simulink model "ASM_Traffic_new"  (R2024a)
settings: Solver=ode1  StartTime=SIM.tstart.v  StopTime=SIM.tend.v  FixedStep=SIM.StepSize.v  RelTol=1e-3
PostLoadFcn:
  | if any(exist('dsrtsu_mdlpostloadfcn', 'file') ~= 0), dsrtsu_mdlpostloadfcn('Execute', bdroot); end
  | try, asm_mdl_postloadfcn(bdroot, 'UpdateModel', 3600); catch, disp(lasterr); end,
InitFcn:
  | , if any(exist('rtifpga_mdlclblib', 'file') ~= 0), rtifpga_mdlclblib('Init', bdroot); end,
  | , if any(exist('dsmpb_private', 'file') ~= 0), dsmpb_private('dsmpb_mdlclblib', 'Init', bdroot); end,
undefined symbols (not defined in the file): _to_, a0b2, ASM_BrakeHydraulics_DemoSystems, ASM_VehicleDynamics_DemoSystems, b98103fe8ad365046cd0, BrakeCircuit, CPT, Crankshaft, DiscIntNeverNeededParam, dsmsi, FinalDriveAssembly, MDL, ModeSignals, Pos_BrakePedal_Maneuver, rad, RefSignals, s_to_rpm, SIM, SoftECU, Suspension, Tire, Transmission
libraries: ASM_Traffic_lib x135, simulink x100, ASM_Utils_lib x77, ASM_VehicleDynamics_lib x70, ASM_Environment_lib x22, dsmpblib x20, dsmsilib x15, MDLD_Utils_lib x10, ASM_BrakeHydraulics_lib x3
(part 5 of 63)

== system ASM_Traffic_new/VehicleDynamics/Interface_In ==
  note: Vehicle Dynamics
  In : Inport
  Bus Creator2 : BusCreator  Inputs=3
  Bus Selector : BusSelector  OutputSignals=Environment.Plant.Sw_ModelPortBlocks[0Disabled|1Enabled],Environment.Plant.Sw_ModelDeskPlottingInterface[0Disabled|1Enabled],Engine.Plant.Trq_MeanEff_Engine[Nm],Driver.Plant.Pos_BrakePedal[%],Driver.Plant.Pos_AccPedal[%],Environment.Plant.Reset_States[0|1],Environment.Plant.ECU_Commands[],DomainControl.TorqueManager.Control.Vehicle_Topology[-2|-1|0|2],Drivetrain.Plant.Trq_Shaft[FL;FR;RL;RR][Nm],Environment.Plant.v_Wind_Coor_Sys_E[x;y;z][m|s],Environment.Plant.p_Ambient[Pa],Environment.Plant.T_Ambient[degC],Driver.Plant.Angle_SteeringWheel[deg],Environment.Plant.Trq_Driver_External[Nm],Environment.Plant.Pos_z_CP[:][m],Environment.Plant.Fric_Coeff_CP[:][],Environment.Plant.UnitVec_z_CP[:][x;y;z],Environment.Plant.Sw_Tire_Parameter_Set_CP[:][1|2|3|4],Environment.Plant.Sw_ParkingBrake[0Off|1On],Environment.Plant.Sw_SteeringMode[1Angle|2Trq],Environment.Plant.Keep_VehiclePosition[0|1],Environment.Plant.Pos_Vehicle_Init_CoorSys_E[x;y;z][m],Environment.Plant.Angle_Vehicle_Init_CoorSys_E[x;y;z][rad],Environment.Plant.q_dt_Vehicle_Init[6x1],Environment.Plant.Sw_Steering_Mode[1Manual|2ManSched],Environment.Plant.Const_Steering_Mode_Manual[1Angle|2Trq],DomainControl.StartSystem.Control.Sw_Ignition[0|1],DomainControl.DriverAssistance.Control.Enable_Trq_Decrease_ACC[0|1],DomainControl.DriverAssistance.Control.Trq_DecreaseRequest_ACC[Nm],DomainControl.TorqueManager.Control.Trq_Request_Brake[Nm]
  Bus Selector1 : BusSelector  OutputSignals=Environment.Plant.Sw_ModelPortBlocks[0Disabled|1Enabled]
  ExternalSignals : Subsystem
  M_Articulated_T[1x36] : Constant  Value=zeros(1,36)
  ModelSignals : Subsystem
  Q_Articulated_T[6x1] : Constant  Value=[0; 0; 0; 0; 0; 0]
  Trq[Nm] : Constant  Value=0
  Trq_Hitch_CoorSys_V[x;y;z][Nm] : Constant  Value=[0 0 0]
  Out : Outport  VectorParamsAs1DForOutWhenUnconnected=off
  wires:
  Bus Selector1/1 -> ExternalSignals/Enable  "<Sw_ModelPortBlocks[0Disabled|1Enabled]>"
  ExternalSignals/2(ExternalPlant) -> Bus Creator2/3
  ExternalSignals/1(ExternalECU) -> Bus Creator2/2
  Bus Creator2/1 -> Out/1
  ModelSignals/1(Out) -> Bus Creator2/1
  Trq[Nm]/1 -> ModelSignals/31(Trq_EM_Front[Nm])
  Q_Articulated_T[6x1]/1 -> ModelSignals/32(Q_Articulated_T[6x1])
  Trq_Hitch_CoorSys_V[x;y;z][Nm]/1 -> ModelSignals/33(Trq_Hitch_CoorSys_V[x;y;z][Nm])
  M_Articulated_T[1x36]/1 -> ModelSignals/34(M_Articulated_T[1x36])
  Bus Selector/1 -> ModelSignals/1(Sw_ModelPortBlocks[0Disabled|1Enabled])  "<Sw_ModelPortBlocks[0Disabled|1Enabled]>"
  Bus Selector/2 -> ModelSignals/2(Sw_ModelDeskPlottingInterface[0Disabled|1Enabled])  "<Sw_ModelDeskPlottingInterface[0Disabled|1Enabled]>"
  Bus Selector/3 -> ModelSignals/3(Trq_Eff_Engine[Nm])  "<Trq_MeanEff_Engine[Nm]>"
  Bus Selector/4 -> ModelSignals/4(Pos_BrakePedal[%])  "<Pos_BrakePedal[%]>"
  Bus Selector/5 -> ModelSignals/5(Pos_AccPedal[%])  "<Pos_AccPedal[%]>"
  Bus Selector/6 -> ModelSignals/6(Reset_VehicleStates[0|1])  "<Reset_States[0|1]>"
  Bus Selector/7 -> ModelSignals/7(ECU_Commands[])  "<ECU_Commands[]>"
  Bus Selector/8 -> ModelSignals/8(Vehicle_Topology[-2|-1|0|2])  "<Vehicle_Topology[-2|-1|0|2]>"
  Bus Selector/9 -> ModelSignals/9(Trq_Shaft[FL,FR,RL,RR][Nm])  "<Trq_Shaft[FL;FR;RL;RR][Nm]>"
  Bus Selector/10 -> ModelSignals/10(v_Wind_Coor_Sys_E[x;y;z][m|s])  "<v_Wind_Coor_Sys_E[x;y;z][m|s]>"
  Bus Selector/11 -> ModelSignals/11(p_Ambient[Pa])  "<p_Ambient[Pa]>"
  Bus Selector/12 -> ModelSignals/12(T_Ambient[degC])  "<T_Ambient[degC]>"
  Bus Selector/13 -> ModelSignals/13(Angle_SteeringWheel[deg])  "<Angle_SteeringWheel[deg]>"
  Bus Selector/14 -> ModelSignals/14(Trq_Driver_External[Nm])  "<Trq_Driver_External[Nm]>"
  Bus Selector/15 -> ModelSignals/15(Pos_z_CP[FL;FR;RL;RR][m])  "<Pos_z_CP[:][m]>"
  Bus Selector/16 -> ModelSignals/16(Fric_Coeff_CP[FL;FR;RL;RR][])  "<Fric_Coeff_CP[:][]>"
  Bus Selector/17 -> ModelSignals/17(UnitVec_z_CP[FL;FR;RL;RR][x;y;z])  "<UnitVec_z_CP[:][x;y;z]>"
  Bus Selector/18 -> ModelSignals/18(Sw_Tire_Parameter_Set_CP[FL;FR;RL;RR][1|2|3|4])  "<Sw_Tire_Parameter_Set_CP[:][1|2|3|4]>"
  Bus Selector/19 -> ModelSignals/19(Sw_ParkingBrake[0Off|1On])  "<Sw_ParkingBrake[0Off|1On]>"
  Bus Selector/20 -> ModelSignals/20(Sw_SteeringMode[1Angle|2Trq])  "<Sw_SteeringMode[1Angle|2Trq]>"
  Bus Selector/21 -> ModelSignals/21(Keep_VehiclePosition[0|1])  "<Keep_VehiclePosition[0|1]>"
  Bus Selector/22 -> ModelSignals/22(Pos_Vehicle_Init_CoorSys_E[x;y;z][m])  "<Pos_Vehicle_Init_CoorSys_E[x;y;z][m]>"
  Bus Selector/23 -> ModelSignals/23(Angle_Vehicle_Init_CoorSys_E[x;y;z][rad])  "<Angle_Vehicle_Init_CoorSys_E[x;y;z][rad]>"
  Bus Selector/24 -> ModelSignals/24(q_dt_Vehicle_Init[6x1])  "<q_dt_Vehicle_Init[6x1]>"
  Bus Selector/25 -> ModelSignals/25(Sw_Steering_Mode[1Manual|2ManSched])  "<Sw_Steering_Mode[1Manual|2ManSched]>"
  Bus Selector/26 -> ModelSignals/26(Const_Steering_Mode_Manual[1Angle|2Trq])  "<Const_Steering_Mode_Manual[1Angle|2Trq]>"
  Bus Selector/27 -> ModelSignals/27(Sw_Ignition[0Off|1On])  "<Sw_Ignition[0|1]>"
  Bus Selector/28 -> ModelSignals/28(Enable_Trq_Brake_Extern[0|1])  "<Enable_Trq_Decrease_ACC[0|1]>"
  Bus Selector/29 -> ModelSignals/29(Trq_Brake_Request_Extern[Nm])  "<Trq_DecreaseRequest_ACC[Nm]>"
  Bus Selector/30 -> ModelSignals/30(Trq_Request_Brake[Nm])  "<Trq_Request_Brake[Nm]>"
  In/1 -> Bus Selector/1, Bus Selector1/1

== system ASM_Traffic_new/VehicleDynamics/Interface_Out ==
  note: VehicleDynamics
  In : Inport
  Active_CP_VehDyn[] : Constant  Value=[1,2,3,4,5,6,9,10]
  Animation : Subsystem
  Bus Creator2 : BusCreator  Inputs=3
  Bus Selector1 : BusSelector  OutputSignals=Control.ECU_Brake.ECU_Mode.ECU_ESP_Mode[0None|1ABS|2ESP|3ASR],Control.ECU_Brake.DesiredPressure.Enable_p_Brake_Desired[0|1],Control.ECU_Brake.DesiredPressure.p_Brake_Desired[bar],Control.ECU_Brake.ESP_Trq_Intervention.Enable_TrqDecrease_Fast_ESP[0|1],Control.ECU_Brake.ESP_Trq_Intervention.Trq_DecreaseRequest_Fast_ESP[Nm],Control.ECU_Brake.ESP_Trq_Intervention.Enable_TrqDecrease_Slow_ESP[0|1],Control.ECU_Brake.ESP_Trq_Intervention.Trq_DecreaseRequest_Slow_ESP[Nm],Control.ECU_Brake.ESP_Trq_Intervention.Enable_TrqIncrease_ESP[0|1],Control.ECU_Brake.ESP_Trq_Intervention.Trq_IncreaseRequest_ESP[Nm]
  Bus Selector4 : BusSelector  OutputSignals=Plant.VehicleDynamics.Wheel.WheelSpeed2.omega_Mean_Wheel[rad|s],Plant.VehicleDynamics.Wheel.WheelSpeed2.omega_Wheel[FL;FR;RL;RR][rad|s],Plant.VehicleDynamics.VehicleMovement.Velocities.Vehicle.Linear.v_Total_Vehicle[km|h],Plant.VehicleDynamics.VehicleMovement.Velocities.Generalized.v_Vehicle[x;y;z][km|h],Plant.VehicleDynamics.VehicleMovement.VehicleEquationOfMotion.GeneralizedVelocitiesDerivative.v_Vehicle_dt[x;y;z][m|s2],Plant.VehicleDynamics.VehicleMovement.SensorMotion.Sensor1.a_Sensor1_CoorSys_V[x;y;z][m|s2],Plant.VehicleDynamics.VehicleMovement.Velocities.Generalized.w_Vehicle[x;y;z][deg|s],Plant.VehicleDynamics.VehicleMovement.VehicleEquationOfMotion.GeneralizedVelocitiesDerivative.w_Vehicle_dt[x;y;z][rad|s2],Plant.VehicleDynamics.Tire.Tire_allSignals.Tire_FL.ContactPoint.Pos_CP_CoorSys_E[x;y][m],Plant.VehicleDynamics.Tire.Tire_allSignals.Tire_FR.ContactPoint.Pos_CP_CoorSys_E[x;y][m],Plant.VehicleDynamics.Tire.Tire_allSignals.Tire_RL.ContactPoint.Pos_CP_CoorSys_E[x;y][m],Plant.VehicleDynamics.Tire.Tire_allSignals.Tire_RR.ContactPoint.Pos_CP_CoorSys_E[x;y][m],Plant.VehicleDynamics.Steering.i_Steering_Mean[],Plant.VehicleDynamics.Steering.Angle_SteeringWheel[deg],Plant.VehicleDynamics.Steering.Angle_SteeringWheel_dt[deg|s],Plant.VehicleDynamics.Steering.ForcesAndTorques.Trq_Steering[Nm],Plant.VehicleDynamics.Tire.r_Dyn_Tire[FL;FR;RL;RR][m],Plant.VehicleDynamics.Tire.Coef_RollingRes[FL;FR;RL;RR][],Plant.VehicleDynamics.Tire.CorneringStiffness[FL;FR;RL;RR][N|rad],Plant.VehicleDynamics.VehicleMovement.Positions.Vehicle.Linear.Pos_Vehicle_CoorSys_E[m],Plant.VehicleDynamics.VehicleMovement.Positions.Vehicle.Angular.Angle_V[Alpha;Beta;Gamma][deg],Plant.VehicleDynamics.VehicleMovement.Positions.Vehicle.Linear.s_Vehicle[m],Plant.VehicleDynamics.VehicleMovement.Velocities.Vehicle.Linear.v_Vehicle_CoG[x;y;z][km|h].v_x_Vehicle_CoG[km|h],Plant.VehicleDynamics.VehicleMovement.Velocities.Vehicle.Linear.v_Vehicle_CoG[x;y;z][km|h].v_y_Vehicle_CoG[km|h],Plant.VehicleDynamics.VehicleMovement.Velocities.Vehicle.Linear.v_Vehicle_CoG[x;y;z][km|h].v_z_Vehicle_CoG[km|h],Plant.VehicleDynamics.VehicleMovement.Velocities.Vehicle.Angular.w_Vehicle_CoG[x;y;z][deg|s].RollRate_Vehicle_CoG[deg|s],Plant.VehicleDynamics.VehicleMovement.Velocities.Vehicle.Angular.w_Vehicle_CoG[x;y;z][deg|s].PitchRate_Vehicle_CoG[deg|s],Plant.VehicleDynamics.VehicleMovement.Velocities.Vehicle.Angular.w_Vehicle_CoG[x;y;z][deg|s].YawRate_Vehicle_CoG[deg|s],Plant.VehicleDynamics.VehicleMovement.Accelerations.VehicleCoG.Linear.a_Vehicle_CoG[x;y;z][m|s2].a_x_Vehicle_CoG[m|s2],Plant.VehicleDynamics.VehicleMovement.Accelerations.VehicleCoG.Linear.a_Vehicle_CoG[x;y;z][m|s2].a_y_Vehicle_CoG[m|s2],Plant.VehicleDynamics.VehicleMovement.Accelerations.VehicleCoG.Linear.a_Vehicle_CoG[x;y;z][m|s2].a_z_Vehicle_CoG[m|s2],Plant.VehicleDynamics.VehicleMovement.Accelerations.VehicleCoG.Angular.w_Vehicle_CoG_dt[x;y;z][rad|s2].w_x_Vehicle_CoG_dt[rad|s2],Plant.VehicleDynamics.VehicleMovement.Accelerations.VehicleCoG.Angular.w_Vehicle_CoG_dt[x;y;z][rad|s2].w_y_Vehicle_CoG_dt[rad|s2],Plant.VehicleDynamics.VehicleMovement.Accelerations.VehicleCoG.Angular.w_Vehicle_CoG_dt[x;y;z][rad|s2].w_z_Vehicle_CoG_dt[rad|s2],Plant.VehicleDynamics.VehicleMovement.VehicleMassAndAdditionalLoads.m_TotalVehicle[kg],Plant.VehicleDynamics.VehicleMovement.VehicleMassAndAdditionalLoads.Pos_x_CoG_Vehicle_Total[m],Plant.VehicleDynamics.VehicleMovement.VehicleMassAndAdditionalLoads.Inertia_z_Vehicle_Total[kgm2],Plant.VehicleDynamics.Aerodynamics.Forces.F_x_Aero_CoorSys_V[N],Plant.VehicleDynamics.Aerodynamics.Coefficients.Cw_x[],Plant.VehicleDynamics.VehicleMovement.MassForcesAndTorques.GravitationalForces.F_Vehicle_Gravitational[x;y;z][N],Plant.VehicleDynamics.VehicleMovement.Positions.Vehicle.Angular.RotationMatrix_V_to_E[1x9],Plant.VehicleDynamics.VehicleMovement.Positions.Vehicle.Angular.RotationMatrix_V_to_E_T[1x9],Plant.VehicleDynamics.Suspension.SuspensionFront.RelativePositionFront.Pos_Wheel[FL;FR][x;y;z][m].Pos_FL_Wheel[x;y;z][m],Plant.VehicleDynamics.Suspension.SuspensionFront.RelativePositionFront.Pos_Wheel[FL;FR][x;y;z][m].Pos_FR_Wheel[x;y;z][m],Plant.VehicleDynamics.Suspension.SuspensionRear.RelativePositionRear.Pos_Wheel[RL;RR][x;y;z][m].Pos_RL_Wheel[x;y;z][m],Plant.VehicleDynamics.Suspension.SuspensionRear.RelativePositionRear.Pos_Wheel[RL;RR][x;y;z][m].Pos_RR_Wheel[x;y;z][m],Plant.VehicleDynamics.Brake.BrakeDisc.MaximumTorque.Trq_Max_Brake[Nm],Plant.VehicleDynamics.Tire.Const_r_unloaded_Tire_Mean[m],Plant.VehicleDynamics.Tire.CorneringStiffness_Tire_Front[N|rad],Plant.VehicleDynamics.Tire.CorneringStiffness_Tire_Rear[N|rad],Plant.VehicleDynamics.Tire.Coef_RollingRes_Mean[],Plant.VehicleDynamics.VehicleMovement.Positions.Vehicle.Linear.Pos_Vehicle_CoorSys_E[x;y;z][m].Pos_x_Vehicle_CoorSys_E[m],Plant.VehicleDynamics.VehicleMovement.Positions.Vehicle.Linear.Pos_Vehicle_CoorSys_E[x;y;z][m].Pos_y_Vehicle_CoorSys_E[m],Plant.VehicleDynamics.VehicleMovement.Positions.Vehicle.Angular.Angle_Vehicle_CoorSys_E[x;y;z][deg].Angle_Yaw_Vehicle_CoorSys_E[deg],Plant.VehicleDynamics.DrivingResistances.F_Driving_Res[N],Plant.VehicleDynamics.Brake.MasterBrakeCylinder.Sw_MasterBrakeCylinder_Mode[1linear|2physical|3Booster|4BrakeByWire],Plant.UserInterface.Suspension.Sw_Rotation[1Cardan|2ToeCamberCaster],Plant.UserInterface.Tire.Tire.Sw_r_Tire[1:intern;2:extern],Plant.UserInterface.Tire.Tire.r_Tire_extern[m],Plant.VehicleDynamics.Wheel.WheelSpeed2.omega_Wheel[FL;FR;RL;RR][rad|s],Plant.VehicleDynamics.Tire.Slip_x_Wheel[]
  Control_ModelSignals : Subsystem
  Plant_ModelSignals : Subsystem
  Pos_CP_Front_CoorSys_E[x;y][m] : Constant  Value=[0;0]
  Pos_CP_R2L2_CoorSys_E[x;y][m] : Constant  Value=[0;0]
  Pos_CP_R2L_CoorSys_E[x;y][m] : Constant  Value=[0;0]
  Pos_CP_R2R2_CoorSys_E[x;y][m] : Constant  Value=[0;0]
  Pos_CP_R2R_CoorSys_E[x;y][m] : Constant  Value=[0;0]
  Pos_CP_RL2_CoorSys_E[x;y][m] : Constant  Value=[0;0]
  Pos_CP_RR2_CoorSys_E[x;y][m] : Constant  Value=[0;0]
  Pos_CP_Rear_CoorSys_E[x;y][m] : Constant  Value=[0;0]
  Out : Outport  VectorParamsAs1DForOutWhenUnconnected=off
  wires:
  Bus Selector4/46 -> Plant_ModelSignals/46(Pos_RR_Wheel[x;y;z][m])  "<Pos_RR_Wheel[x;y;z][m]>"
  Bus Selector4/45 -> Plant_ModelSignals/45(Pos_RL_Wheel[x;y;z][m])  "<Pos_RL_Wheel[x;y;z][m]>"
  Bus Selector4/34 -> Plant_ModelSignals/34(w_z_Vehicle_CoG_dt[rad|s])  "<w_z_Vehicle_CoG_dt[rad|s2]>"
  Bus Selector4/33 -> Plant_ModelSignals/33(w_y_Vehicle_CoG_dt[rad|s])  "<w_y_Vehicle_CoG_dt[rad|s2]>"
  Bus Selector4/32 -> Plant_ModelSignals/32(w_x_Vehicle_CoG_dt[rad|s])  "<w_x_Vehicle_CoG_dt[rad|s2]>"
  Bus Selector4/31 -> Plant_ModelSignals/31(a_z_Vehicle_CoG[m|s2])  "<a_z_Vehicle_CoG[m|s2]>"
  Bus Selector4/29 -> Plant_ModelSignals/29(a_x_Vehicle_CoG[m|s2])  "<a_x_Vehicle_CoG[m|s2]>"
  Bus Selector4/27 -> Plant_ModelSignals/27(PitchRate_Vehicle_CoG[deg|s])  "<PitchRate_Vehicle_CoG[deg|s]>"
  Bus Selector4/25 -> Plant_ModelSignals/25(v_z_Vehicle_CoG[km|h])  "<v_z_Vehicle_CoG[km|h]>"
  Bus Selector4/6 -> Plant_ModelSignals/6(a_Vehicle[x;y;z][m|s2])  "<a_Sensor1_CoorSys_V[x;y;z][m|s2]>"
  Pos_CP_Rear_CoorSys_E[x;y][m]/1 -> Plant_ModelSignals/70(Pos_CP_Rear_CoorSys_E[x;y][m])
  Pos_CP_Front_CoorSys_E[x;y][m]/1 -> Plant_ModelSignals/69(Pos_CP_Front_CoorSys_E[x;y][m])
  In/1 -> Bus Selector1/1, Bus Selector4/1, Animation/1(In)
  Bus Selector4/1 -> Plant_ModelSignals/1(omega_Mean_Wheel[rad|s])  "<omega_Mean_Wheel[rad|s]>"
  Bus Selector4/2 -> Plant_ModelSignals/2(omega_Wheel[FL;FR;RL;RR][rad|s])  "<omega_Wheel[FL;FR;RL;RR][rad|s]>"
  Bus Selector4/3 -> Plant_ModelSignals/3(v_Vehicle[km|h])  "<v_Total_Vehicle[km|h]>"
  Bus Selector4/51 -> Plant_ModelSignals/51(Coef_RollingRes_Mean[])  "<Coef_RollingRes_Mean[]>"
  Bus Selector4/50 -> Plant_ModelSignals/50(CorneringStiffness_Tire_Rear[N|rad])  "<CorneringStiffness_Tire_Rear[N|rad]>"
  Bus Selector4/49 -> Plant_ModelSignals/49(CorneringStiffness_Tire_Front[N|rad])  "<CorneringStiffness_Tire_Front[N|rad]>"
  Bus Selector4/48 -> Plant_ModelSignals/48(Const_r_unloaded_Tire_Mean[m])  "<Const_r_unloaded_Tire_Mean[m]>"
  Bus Selector4/47 -> Plant_ModelSignals/47(Trq_Max_Brake[Nm])  "<Trq_Max_Brake[Nm]>"
  Bus Selector4/44 -> Plant_ModelSignals/44(Pos_FR_Wheel[x;y;z][m])  "<Pos_FR_Wheel[x;y;z][m]>"
  Bus Selector4/43 -> Plant_ModelSignals/43(Pos_FL_Wheel[x;y;z][m])  "<Pos_FL_Wheel[x;y;z][m]>"
  Bus Selector4/42 -> Plant_ModelSignals/42(RotationMatrix_V_to_E_T[1x9])  "<RotationMatrix_V_to_E_T[1x9]>"
  Bus Selector4/41 -> Plant_ModelSignals/41(RotationMatrix_V_to_E[1x9])  "<RotationMatrix_V_to_E[1x9]>"
  Bus Selector4/40 -> Plant_ModelSignals/40(F_Vehicle_Gravitational[x;y;z][N])  "<F_Vehicle_Gravitational[x;y;z][N]>"
  Bus Selector4/39 -> Plant_ModelSignals/39(Cw_x[])  "<Cw_x[]>"
  Bus Selector4/38 -> Plant_ModelSignals/38(F_x_Aero_CoorSys_V[N])  "<F_x_Aero_CoorSys_V[N]>"
  Bus Selector4/37 -> Plant_ModelSignals/37(Inertia_z_Vehicle_Total[kgm2])  "<Inertia_z_Vehicle_Total[kgm2]>"
  Bus Selector4/36 -> Plant_ModelSignals/36(Pos_x_CoG_Vehicle_Total[m])  "<Pos_x_CoG_Vehicle_Total[m]>"
  Bus Selector4/35 -> Plant_ModelSignals/35(m_TotalVehicle[kg])  "<m_TotalVehicle[kg]>"
  Bus Selector4/30 -> Plant_ModelSignals/30(a_y_Vehicle_CoG[m|s2])  "<a_y_Vehicle_CoG[m|s2]>"
  Bus Selector4/28 -> Plant_ModelSignals/28(YawRate_Vehicle_CoG[deg|s])  "<YawRate_Vehicle_CoG[deg|s]>"
  Bus Selector4/26 -> Plant_ModelSignals/26(RollRate_Vehicle_CoG[deg|s])  "<RollRate_Vehicle_CoG[deg|s]>"
  Bus Selector4/24 -> Plant_ModelSignals/24(v_y_Vehicle_CoG[km|h])  "<v_y_Vehicle_CoG[km|h]>"
  Bus Selector4/23 -> Plant_ModelSignals/23(v_x_Vehicle_CoG[km|h])  "<v_x_Vehicle_CoG[km|h]>"
  Bus Selector4/22 -> Plant_ModelSignals/22(s_Vehicle[m])  "<s_Vehicle[m]>"
  Bus Selector4/21 -> Plant_ModelSignals/21(Angle_Vehicle_CoorSys_E[x;y;z][deg])  "<Angle_V[Alpha;Beta;Gamma][deg]>"
  Bus Selector4/20 -> Plant_ModelSignals/20(Pos_Vehicle_CoorSys_E[x;y;z][m])  "<Pos_Vehicle_CoorSys_E[m]>"
  Bus Selector4/19 -> Plant_ModelSignals/19(CorneringStiffness[FL;FR;RL;RR][N])  "<CorneringStiffness[FL;FR;RL;RR][N|rad]>"
  Bus Selector4/18 -> Plant_ModelSignals/18(Coef_RollingRes[FL;FR;RL;RR][])  "<Coef_RollingRes[FL;FR;RL;RR][]>"
  Bus Selector4/17 -> Plant_ModelSignals/17(r_Dyn_Tire[FL;FR;RL;RR][m])  "<r_Dyn_Tire[FL;FR;RL;RR][m]>"
  Bus Selector4/16 -> Plant_ModelSignals/16(Trq_SteeringWheel[Nm])  "<Trq_Steering[Nm]>"
  Bus Selector4/14 -> Plant_ModelSignals/14(Angle_SteeringWheel[deg])  "<Angle_SteeringWheel[deg]>"
  Bus Selector4/13 -> Plant_ModelSignals/13(i_Steering_Mean[])  "<i_Steering_Mean[]>"
  Bus Selector4/12 -> Plant_ModelSignals/12(Pos_CP_RR_CoorSys_E[x;y][m])  "<Pos_CP_CoorSys_E[x;y][m]>"
  Bus Selector4/11 -> Plant_ModelSignals/11(Pos_CP_RL_CoorSys_E[x;y][m])  "<Pos_CP_CoorSys_E[x;y][m]>"
  Bus Selector4/10 -> Plant_ModelSignals/10(Pos_CP_FR_CoorSys_E[x;y][m])  "<Pos_CP_CoorSys_E[x;y][m]>"
  Bus Selector4/9 -> Plant_ModelSignals/9(Pos_CP_FL_CoorSys_E[x;y][m])  "<Pos_CP_CoorSys_E[x;y][m]>"
  Bus Selector4/8 -> Plant_ModelSignals/8(w_Vehicle_dt[x;y;z][rad|s2])  "<w_Vehicle_dt[x;y;z][rad|s2]>"
  Bus Selector4/7 -> Plant_ModelSignals/7(w_Vehicle[x;y;z][deg|s])  "<w_Vehicle[x;y;z][deg|s]>"
  Bus Selector4/5 -> Plant_ModelSignals/5(v_Vehicle_dt[x;y;z][m|s2])  "<v_Vehicle_dt[x;y;z][m|s2]>"
  Bus Selector4/4 -> Plant_ModelSignals/4(v_Vehicle[x;y;z][km|h])  "<v_Vehicle[x;y;z][km|h]>"
  Bus Selector4/52 -> Plant_ModelSignals/52(Pos_x_Vehicle_CoorSys_E[m])  "<Pos_x_Vehicle_CoorSys_E[m]>"
  Bus Selector4/53 -> Plant_ModelSignals/53(Pos_y_Vehicle_CoorSys_E[m])  "<Pos_y_Vehicle_CoorSys_E[m]>"
  Bus Selector4/54 -> Plant_ModelSignals/54(Angle_Yaw_Vehicle_CoorSys_E[deg])  "<Angle_Yaw_Vehicle_CoorSys_E[deg]>"
  Bus Selector4/55 -> Plant_ModelSignals/55(F_Driving_Res[N])  "<F_Driving_Res[N]>"
  Pos_CP_RL2_CoorSys_E[x;y][m]/1 -> Plant_ModelSignals/62(Pos_CP_RL2_CoorSys_E[x;y][m])
  Pos_CP_RR2_CoorSys_E[x;y][m]/1 -> Plant_ModelSignals/63(Pos_CP_RR2_CoorSys_E[x;y][m])
  Pos_CP_R2L_CoorSys_E[x;y][m]/1 -> Plant_ModelSignals/64(Pos_CP_R2L_CoorSys_E[x;y][m])
  Pos_CP_R2L2_CoorSys_E[x;y][m]/1 -> Plant_ModelSignals/65(Pos_CP_R2L2_CoorSys_E[x;y][m])
  Pos_CP_R2R_CoorSys_E[x;y][m]/1 -> Plant_ModelSignals/66(Pos_CP_R2R_CoorSys_E[x;y][m])
  Pos_CP_R2R2_CoorSys_E[x;y][m]/1 -> Plant_ModelSignals/67(Pos_CP_R2R2_CoorSys_E[x;y][m])
  Active_CP_VehDyn[]/1 -> Plant_ModelSignals/68(Active_CP_VehDyn[])
  Bus Selector1/3 -> Control_ModelSignals/3(p_Brake_Desired[bar])  "<p_Brake_Desired[bar]>"
  Bus Selector1/5 -> Control_ModelSignals/5(Trq_DecreaseRequest_Fast_ESP[Nm])  "<Trq_DecreaseRequest_Fast_ESP[Nm]>"
  Bus Selector1/1 -> Control_ModelSignals/1(ECU_ESP_Mode[0None|1ABS|2ESP|3ASR])  "<ECU_ESP_Mode[0None|1ABS|2ESP|3ASR]>"
  Bus Selector1/6 -> Control_ModelSignals/6(Enable_TrqDecrease_Slow_ESP[0|1])  "<Enable_TrqDecrease_Slow_ESP[0|1]>"
  Bus Selector1/2 -> Control_ModelSignals/2(Enable_p_Brake_Desired[0|1])  "<Enable_p_Brake_Desired[0|1]>"
  Bus Selector1/4 -> Control_ModelSignals/4(Enable_TrqDecrease_Fast_ESP[0|1])  "<Enable_TrqDecrease_Fast_ESP[0|1]>"
  Bus Selector1/8 -> Control_ModelSignals/8(Enable_TrqIncrease_ESP[0|1])  "<Enable_TrqIncrease_ESP[0|1]>"
  Bus Selector1/7 -> Control_ModelSignals/7(Trq_DecreaseRequest_Slow_ESP[Nm])  "<Trq_DecreaseRequest_Slow_ESP[Nm]>"
  Bus Selector1/9 -> Control_ModelSignals/9(Trq_IncreaseRequest_ESP[Nm])  "<Trq_IncreaseRequest_ESP[Nm]>"
  Bus Creator2/1 -> Out/1  "VehicleDynamics"
  Control_ModelSignals/1(Out) -> Bus Creator2/1
  Bus Selector4/56 -> Plant_ModelSignals/56(Sw_MasterBrakeCylinder_Mode[1linear|2physical|3Booster])  "<Sw_MasterBrakeCylinder_Mode[1linear|2physical|3Booster|4BrakeByWire]>"
  Bus Selector4/57 -> Plant_ModelSignals/57(Sw_Rotation[1Cardan|2ToeCamberCaster])  "<Sw_Rotation[1Cardan|2ToeCamberCaster]>"
  Bus Selector4/58 -> Plant_ModelSignals/58(Sw_r_Tire[1:intern;2:extern])  "<Sw_r_Tire[1:intern;2:extern]>"
  Bus Selector4/59 -> Plant_ModelSignals/59(r_Tire_extern[m])  "<r_Tire_extern[m]>"
  Plant_ModelSignals/1(Out) -> Bus Creator2/2
  Animation/1(Out) -> Bus Creator2/3
  Bus Selector4/15 -> Plant_ModelSignals/15(Angle_SteeringWheel_dt[deg|s])  "<Angle_SteeringWheel_dt[deg|s]>"
  Bus Selector4/60 -> Plant_ModelSignals/60(omega_Wheel[rad|s])  "<omega_Wheel[FL;FR;RL;RR][rad|s]>"
  Bus Selector4/61 -> Plant_ModelSignals/61(Slip_x_Wheel[])  "<Slip_x_Wheel[]>"

== system ASM_Traffic_new/VehicleDynamics/Plant ==
  note: Vehicle Dynamics
  Interface_In : Inport
  Control : Inport  Port=2
  Bus Creator : BusCreator  Inputs=2
  Sw_Plant_Signals : Subsystem
  UserInterface : Subsystem
  VehicleDynamics : Subsystem
  Plant : Outport  VectorParamsAs1DForOutWhenUnconnected=off
  wires:
  Bus Creator/1 -> Plant/1  "Plant"
  UserInterface/1(Out) -> Bus Creator/2, VehicleDynamics/1(UserInterface)
  VehicleDynamics/2(PlantModel_Signals) -> Sw_Plant_Signals/1(PlantModel_Signals)
  Interface_In/1 -> Sw_Plant_Signals/2(ExternalPlant_Signals), VehicleDynamics/2(Interface_In)
  Sw_Plant_Signals/1(Plant_Signals) -> VehicleDynamics/4(Plant_Signals)
  Control/1 -> VehicleDynamics/3(Control)
  VehicleDynamics/1(ASMSignalBus) -> Bus Creator/1, UserInterface/1(In)

== system ASM_Traffic_new/VehicleDynamics/SignalInterface ==
  In : Inport
  ASMSignalInterface : Subsystem  mask(ASM_SIGNAL_INTERFACE){LabelTextfield=VehicleDynamics}
      mask prompts: LabelTextfield "Label"
      mask help:
      | The ASMSignalInterface block processes the ASMSignalBus and provides a vector-based interface for each signal (e.g. ModelDesk Plotting).
      |
      | Always push the update button after you have changed the signal bus structure in order to synchronize the signal interface. The update may take a few seconds.
      | A modified model must be reloaded in ModelDesk to keep consistency of ModelDesk and simulation model plot signals. Therefore select ''Update Model'' from the ''Simulation Model'' context menu of the ModelDesk Project Navigator.
      settings: AttributesFormatString=Label: %<LabelTextfield>
      settings: CopyFcn=|
      | try
      |  set_param(gcb,'LinkStatus', 'none')
      | catch
      | end
      mask Help: eval(['asm_modelhelp(gcbh,''tool'',''ASM_Utils_lib'', ''ASMSIGNALINTERFACE'')'])
      mask DialogControl Hint Prompt: For changes of Label first apply change and then push "Update".
      mask DialogControl UpdateButton Prompt: Update
      mask DialogControl UpdateButton Callback: asm_mdld_plot_block_update(bdroot(gcb), 'update', 'current');
      mask DialogControl UpdateAllButton Prompt: Update All
      mask DialogControl UpdateAllButton Callback: asm_mdld_plot_block_update(bdroot(gcb), 'update', 'all');
  Bus Creator : BusCreator  Inputs=2
  Bus Selector Disable Signals : BusSelector  OutputSignals=ExternalModel.Sw_ModelPortBlocks[0Disabled|1Enabled],ExternalModel.Sw_ModelDeskPlottingInterface[0Disabled|1Enabled]
  ExternalOutports : Subsystem  TreatAsAtomicUnit=on
  wires:
  Bus Selector Disable Signals/2 -> ASMSignalInterface/Enable  "<Sw_ModelDeskPlottingInterface[0Disabled|1Enabled]>"
  Bus Selector Disable Signals/1 -> ExternalOutports/Enable  "<Sw_ModelPortBlocks[0Disabled|1Enabled]>"
  In/1 -> Bus Selector Disable Signals/1
  [ASMBUS_VehicleDynamics_Plant] -> Bus Creator/2, ExternalOutports/1(In1)  "Plant"
  [ASMBUS_VehicleDynamics_Control] -> Bus Creator/1  "Control"
  Bus Creator/1 -> ASMSignalInterface/1(ASMSignalBus)

== system ASM_Traffic_new/AnimationInterface/ANIMATION_INTERFACE/ACC_Instruments ==
  DriverAssistance_Animation : Inport
  ACC_Instruments : dsmsilib/dsmsi_simulation_data_objects_BL1  Priority=10001  parameterStr="{\"Version\":1,\"TransformInput\":false,\"EnableInput\":true,\"Objects\":[{\"Name\":\"ACC_State\",\"TypeClass\":{\"Name\":\"Signal\",\"Class\":3,\"SignalProperty\":{\"Description\":null,\"Unit\":null,\"Type\":0,\"Length\":1,\"ObjectsCount\":1},\"TransformationProperty\":null,\"PositionAndScaleProperty\":null,\"PositionProperty\":null},\"Children\":[],\"Oid\":1},{\"Name\":\"ACC_Target_Detected\",\"TypeClass\":{\"Name\":\"Signal\",\"Class\":3,\"SignalProperty\":{\"Description\":null,\"Unit\":null,\"Type\":0,\"Length\":1,\"ObjectsCount\":1},\"TransformationProperty\":null,\"PositionAndScaleProperty\":null,\"PositionProperty\":null},\"Children\":[],\"Oid\":2},{\"Name\":\"ACC_v_Set\",\"TypeClass\":{\"Name\":\"Signal\",\"Class\":3,\"SignalProperty\":{\"Description\":null,\"Unit\":\"km/h\",\"Type\":0,\"Length\":1,\"ObjectsCount\":1},\"TransformationProperty\":null,\"PositionAndScaleProperty\":null,\"PositionProperty\":null},\"Children\":[],\"Oid\":3},{\"Name\":\"ACC_Dist_Set\",\"TypeClass\":{\"Name\":\"Signal\",\"Class\":3,\"SignalProperty\":{\"Description\":null,\"Unit\":\"m\",\"Type\":0,\"Length\":1,\"ObjectsCount\":1},\"TransformationProperty\":null,\"PositionAndScaleProperty\":null,\"PositionProperty\":null},\"Children\":[],\"Oid\":4},{\"Name\":\"ACC_Dist_Target\",\"TypeClass\":{\"Name\":\"Signal\",\"Class\":3,\"SignalProperty\":{\"Description\":null,\"Unit\":\"m\",\"Type\":0,\"Length\":1,\"ObjectsCount\":1},\"TransformationProperty\":null,\"PositionAndScaleProperty\":null,\"PositionProperty\":null},\"Children\":[],\"Oid\":5}]}"  evalStr=dsmsi(gcb, 'EvalJson')  sampleTime=-1  globalBlockId=0  objectsBlockId=dsmsi(gcb, 'GetObjectBlockId')  objectsBlockGuiOpen=dsmsi(gcb, 'GetSdoGuiStatus')  dialogIsOpen=0  blockVersion=60  highPrecision=0  validNameBckp=ACC_Instruments
      settings: SourceProductName=dSPACE MSI Blockset
  Bus Selector7 : BusSelector  OutputSignals=State_ACC[0Off|1On],Target_Detected[0|1],v_Set[km|h],Distance_Set[m],Dist_Long[m]
  Enable_Data_Transfer : Constant
  wires:
  Enable_Data_Transfer/1 -> ACC_Instruments/1
  Bus Selector7/2 -> ACC_Instruments/3  "<Target_Detected[0|1]>"
  Bus Selector7/1 -> ACC_Instruments/2  "<State_ACC[0Off|1On]>"
  Bus Selector7/5 -> ACC_Instruments/6  "<Dist_Long[m]>"
  DriverAssistance_Animation/1 -> Bus Selector7/1
  Bus Selector7/4 -> ACC_Instruments/5  "<Distance_Set[m]>"
  Bus Selector7/3 -> ACC_Instruments/4  "<v_Set[km|h]>"

== system ASM_Traffic_new/AnimationInterface/ANIMATION_INTERFACE/ASM_Vehicle ==
  ASM_Vehicle_Lights : Inport
  VehicleDynamics_Animation : Inport  Port=2
  ASM_Vehicle_Doors : Inport  Port=3
  Chassis : Subsystem
  Demux : Demux  Outputs=6
  Enable_Data_Transfer : Constant
  Pos_y_Offset_Arrow[m] : Constant  Value=0.2
  Pos_z_Offset_Arrow[m] : Constant  Value=0.1
  Scaling_F_Tire[] : Constant  Value=0.0003
  Scaling_Fxy_Arrow[] : Constant  Value=0.5
  Steering_Wheel : Subsystem
  Sw_TireRadius[0|1] : Constant  Value=0
  TireForceLeftFront : Subsystem
  TireForceLeftRear : Subsystem
  TireForceRightFront : Subsystem
  TireForceRightRear : Subsystem
  TireRadius[m] : Constant  Value=0.36
  Vehicle : dsmsilib/dsmsi_simulation_data_objects_BL1  Priority=10001  parameterStr="{\"Version\":1,\"TransformInput\":false,\"EnableInput\":true,\"Objects\":[{\"Oid\":1,\"Name\":\"chassis\",\"TypeClass\":{\"Name\":\"Transformation\",\"Class\":1,\"SignalProperty\":null,\"TransformationProperty\":{\"ObjectsCount\":1,\"TransformMatrixIn\":false,\"TransformMatrixOut\":true,\"AngleInterpretation\":0,\"TransformationOrder\":0,\"RotationOrder\":0,\"TranslationAsParameter\":false,\"Translation\":\"[0 0 0]\",\"RotationAsParameter\":false,\"Rotation\":\"[0 0 0]\",\"ScalingAsParameter\":true,\"Scaling\":\"[1 1 1]\"},\"PositionAndScaleProperty\":null,\"PositionProperty\":null},\"Children\":[{\"Oid\":2,\"Name\":\"steering_wheel\",\"TypeClass\":{\"Name\":\"Transformation\",\"Class\":1,\"SignalProperty\":null,\"TransformationProperty\":{\"ObjectsCount\":1,\"TransformMatrixIn\":false,\"TransformMatrixOut\":false,\"AngleInterpretation\":0,\"TransformationOrder\":0,\"RotationOrder\":0,\"TranslationAsParameter\":false,\"Translation\":\"[0 0 0]\",\"RotationAsParameter\":false,\"Rotation\":\"[0 0 0]\",\"ScalingAsParameter\":true,\"Scaling\":\"[1 1 1]\"},\"PositionAndScaleProperty\":null,\"PositionProperty\":null},\"Children\":[]},{\"Oid\":3,\"Name\":\"wheel_FL\",\"TypeClass\":{\"Name\":\"Transformation\",\"Class\":1,\"SignalProperty\":null,\"TransformationProperty\":{\"ObjectsCount\":1,\"TransformMatrixIn\":false,\"TransformMatrixOut\":false,\"AngleInterpretation\":0,\"TransformationOrder\":0,\"RotationOrder\":1,\"TranslationAsParameter\":false,\"Translation\":\"[0 0 0]\",\"RotationAsParameter\":false,\"Rotation\":\"[0 0 0]\",\"ScalingAsParameter\":false,\"Scaling\":\"[1 1 1]\"},\"PositionAndScaleProperty\":null,\"PositionProperty\":null},\"Children\":[]},{\"Oid\":4,\"Name\":\"wheel_FR\",\"TypeClass\":{\"Name\":\"Transformation\",\"Class\":1,\"SignalProperty\":null,\"TransformationProperty\":{\"ObjectsCount\":1,\"TransformMatrixIn\":false,\"TransformMatrixOut\":false,\"AngleInterpretation\":0,\"TransformationOrder\":0,\"RotationOrder\":1,\"TranslationAsParameter\":false,\"Translation\":\"[0 0 0]\",\"RotationAsParameter\":false,\"Rotation\":\"[0 0 0]\",\"ScalingAsParameter\":false,\"Scaling\":\"[1 1 1]\"},\"PositionAndScaleProperty\":null,\"PositionProperty\":null},\"Children\":[]},{\"Oid\":7,\"Name\":\"wheel_RL\",\"TypeClass\":{\"Name\":\"Transformation\",\"Class\":1,\"SignalProperty\":null,\"TransformationProperty\":{\"ObjectsCount\":1,\"TransformMatrixIn\":false,\"TransformMatrixOut\":false,\"AngleInterpretation\":0,\"TransformationOrder\":0,\"RotationOrder\":1,\"TranslationAsParameter\":false,\"Translation\":\"[0 0 0]\",\"RotationAsParameter\":false,\"Rotation\":\"[0 0 0]\",\"ScalingAsParameter\":false,\"Scaling\":\"[1 1 1]\"},\"PositionAndScaleProperty\":null,\"PositionProperty\":null},\"Children\":[]},{\"Oid\":8,\"Name\":\"wheel_RR\",\"TypeClass\":{\"Name\":\"Transformation\",\"Class\":1,\"SignalProperty\":null,\"TransformationProperty\":{\"ObjectsCount\":1,\"TransformMatrixIn\":false,\"TransformMatrixOut\":false,\"AngleInterpretation\":0,\"TransformationOrder\":0,\"RotationOrder\":1,\"TranslationAsParameter\":false,\"Translation\":\"[0 0 0]\",\"RotationAsParameter\":false,\"Rotation\":\"[0 0 0]\",\"ScalingAsParameter\":false,\"Scaling\":\"[1 1 1]\"},\"PositionAndScaleProperty\":null,\"PositionProperty\":null},\"Children\":[]},{\"Oid\":5,\"Name\":\"_TireFrcs_F_L_x\",\"TypeClass\":{\"Name\":\"Transformation\",\"Class\":1,\"SignalProperty\":null,\"TransformationProperty\":{\"ObjectsCount\":1,\"TransformMatrixIn\":false,\"TransformMatrixOut\":false,\"AngleInterpretation\":0,\"TransformationOrder\":0,\"RotationOrder\":0,\"TranslationAsParameter\":false,\"Translation\":\"[0 0 0]\",\"RotationAsParameter\":true,\"Rotation\":\"[0 90 0]\",\"ScalingAsParameter\":false,\"Scaling\":\"[1 1 1]\"},\"PositionAndScaleProperty\":null,\"PositionProperty\":null},\"Children\":[]},{\"Oid\":12,\"Name\":\"_TireFrcs_F_L_y\",\"TypeClass\":{\"Name\":\"Transformation\",\"Class\":1,\"SignalProperty\":null,\"TransformationProperty\":{\"ObjectsCount\":1,\"TransformMatrixIn\":false,\"TransformMatrixOut\":false,\"AngleInterpretation\":0,\"TransformationOrder\":0,\"RotationOrder\":0,\"TranslationAsParameter\":false,\"Translation\":\"[0 0 0]\",\"RotationAsParameter\":true,\"Rotation\":\"[0 0 -90]\",\"ScalingAsParameter\":false,\"Scaling\":\"[1 1 1]\"},\"PositionAndScaleProperty\":null,\"PositionProperty\":null},\"Children\":[]},{\"Oid\":13,\"Name\":\"_TireFrcs_F_L_z\",\"TypeClass\":{\"Name\":\"Transformation\",\"Class\":1,\"SignalProperty\":null,\"TransformationProperty\":{\"ObjectsCount\":1,\"TransformMatrixIn\":false,\"TransformMatrixOut\":false,\"AngleInterpretation\":0,\"TransformationOrder\":0,\"RotationOrder\":0,\"TranslationAsParameter\":false,\"Translation\":\"[0 0 0]\",\"RotationAsParameter\":true,\"Rotation\":\"[0 0 0]\",\"ScalingAsParameter\":false,\"Scaling\":\"[1 1 1]\"},\"PositionAndScaleProperty\":null,\"PositionProperty\":null},\"Children\":[]},{\"Oid\":6,\"Name\":\"_TireFrcs_F_R_x\",\"TypeClass\":{\"Name\":\"Transformation\",\"Class\":1,\"SignalProperty\":null,\"TransformationProperty\":{\"ObjectsCount\":1,\"TransformMatrixIn\":false,\"TransformMatrixOut\":false,\"AngleInterpretation\":0,\"TransformationOrder\":0,\"RotationOrder\":0,\"TranslationAsParameter\":false,\"Translation\":\"[0 0 0]\",\"RotationAsParameter\":true,\"Rotation\":\"[0 90 0]\",\"ScalingAsParameter\":false,\"Scaling\":\"[1 1 1]\"},\"PositionAndScaleProperty\":null,\"PositionProperty\":null},\"Children\":[]},{\"Oid\":14,\"Name\":\"_TireFrcs_F_R_y\",\"TypeClass\":{\"Name\":\"Transformation\",\"Class\":1,\"SignalProperty\":null,\"TransformationProperty\":{\"ObjectsCount\":1,\"TransformMatrixIn\":false,\"TransformMatrixOut\":false,\"AngleInterpretation\":0,\"TransformationOrder\":0,\"RotationOrder\":0,\"TranslationAsParameter\":false,\"Translation\":\"[0 0 0]\",\"RotationAsParameter\":true,\"Rotation\":\"[0 0 -90]\",\"ScalingAsParameter\":false,\"Scaling\":\"[1 1 1]\"},\"PositionAndScaleProperty\":null,\"PositionProperty\":null},\"Children\":[]},{\"Oid\":15,\"Name\":\"_TireFrcs_F_R_z\",\"TypeClass\":{\"Name\":\"Transformation\",\"Class\":1,\"SignalProperty\":null,\"TransformationProperty\":{\"ObjectsCount\":1,\"TransformMatrixIn\":false,\"TransformMatrixOut\":false,\"AngleInterpretation\":0,\"TransformationOrder\":0,\"RotationOrder\":0,\"TranslationAsParameter\":false,\"Translation\":\"[0 0 0]\",\"RotationAsParameter\":true,\"Rotation\":\"[0 0 0]\",\"ScalingAsParameter\":false,\"Scaling\":\"[1 1 1]\"},\"PositionAndScaleProperty\":null,\"PositionProperty\":null},\"Children\":[]},{\"Oid\":9,\"Name\":\"_TireFrcs_R_L_x\",\"TypeClass\":{\"Name\":\"Transformation\",\"Class\":1,\"SignalProperty\":null,\"TransformationProperty\":{\"ObjectsCount\":1,\"TransformMatrixIn\":false,\"TransformMatrixOut\":false,\"AngleInterpretation\":0,\"TransformationOrder\":0,\"RotationOrder\":0,\"TranslationAsParameter\":false,\"Translation\":\"[0 0 0]\",\"RotationAsParameter\":true,\"Rotation\":\"[0 90 0]\",\"ScalingAsParameter\":false,\"Scaling\":\"[1 1 1]\"},\"PositionAndScaleProperty\":null,\"PositionProperty\":null},\"Children\":[]},{\"Oid\":16,\"Name\":\"_TireFrcs_R_L_y\",\"TypeClass\":{\"Name\":\"Transformation\",\"Class\":1,\"SignalProperty\":null,\"TransformationProperty\":{\"ObjectsCount\":1,\"TransformMatrixIn\":false,\"TransformMatrixOut\":false,\"AngleInterpretation\":0,\"TransformationOrder\":0,\"RotationOrder\":0,\"TranslationAsParameter\":false,\"Translation\":\"[0 0 0]\",\"RotationAsParameter\":true,\"Rotation\":\"[0 0 -90]\",\"ScalingAsParameter\":false,\"Scaling\":\"[1 1 1]\"},\"PositionAndScaleProperty\":null,\"PositionProperty\":null},\"Children\":[]},{\"Oid\":17,\"Name\":\"_TireFrcs_R_L_z\",\"TypeClass\":{\"Name\":\"Transformation\",\"Class\":1,\"SignalProperty\":null,\"TransformationProperty\":{\"ObjectsCount\":1,\"TransformMatrixIn\":false,\"TransformMatrixOut\":false,\"AngleInterpretation\":0,\"TransformationOrder\":0,\"RotationOrder\":0,\"TranslationAsParameter\":false,\"Translation\":\"[0 0 0]\",\"RotationAsParameter\":true,\"Rotation\":\"[0 0 0]\",\"ScalingAsParameter\":false,\"Scaling\":\"[1 1 1]\"},\"PositionAndScaleProperty\":null,\"PositionProperty\":null},\"Children\":[]},{\"Oid\":10,\"Name\":\"_TireFrcs_R_R_x\",\"TypeClass\":{\"Name\":\"Transformation\",\"Class\":1,\"SignalProperty\":null,\"TransformationProperty\":{\"ObjectsCount\":1,\"TransformMatrixIn\":false,\"TransformMatrixOut\":false,\"AngleInterpretation\":0,\"TransformationOrder\":0,\"RotationOrder\":0,\"TranslationAsParameter\":false,\"Translation\":\"[0 0 0]\",\"RotationAsParameter\":true,\"Rotation\":\"[0 90 0]\",\"ScalingAsParameter\":false,\"Scaling\":\"[1 1 1]\"},\"PositionAndScaleProperty\":null,\"PositionProperty\":null},\"Children\":[]},{\"Oid\":18,\"Name\":\"_TireFrcs_R_R_y\",\"TypeClass\":{\"Name\":\"Transformation\",\"Class\":1,\"SignalProperty\":null,\"TransformationProperty\":{\"ObjectsCount\":1,\"TransformMatrixIn\":false,\"TransformMatrixOut\":false,\"AngleInterpretation\":0,\"TransformationOrder\":0,\"RotationOrder\":0,\"TranslationAsParameter\":false,\"Translation\":\"[0 0 0]\",\"RotationAsParameter\":true,\"Rotation\":\"[0 0 -90]\",\"ScalingAsParameter\":false,\"Scaling\":\"[1 1 1]\"},\"PositionAndScaleProperty\":null,\"PositionProperty\":null},\"Children\":[]},{\"Oid\":19,\"Name\":\"_TireFrcs_R_R_z\",\"TypeClass\":{\"Name\":\"Transformation\",\"Class\":1,\"SignalProperty\":null,\"TransformationProperty\":{\"ObjectsCount\":1,\"TransformMatrixIn\":false,\"TransformMatrixOut\":false,\"AngleInterpretation\":0,\"TransformationOrder\":0,\"RotationOrder\":0,\"TranslationAsParameter\":false,\"Translation\":\"[0 0 0]\",\"RotationAsParameter\":true,\"Rotation\":\"[0 0 0]\",\"ScalingAsParameter\":false,\"Scaling\":\"[1 1 1]\"},\"PositionAndScaleProperty\":null,\"PositionProperty\":null},\"Children\":[]},{\"Oid\":11,\"Name\":\"ASM_Vehicle_Lights\",\"TypeClass\":{\"Name\":\"Signal\",\"Class\":3,\"SignalProperty\":{\"ObjectsCount\":1,\"InstrumentInput\":\"Input port\",\"Description\":null,\"Unit\":null,\"Type\":7,\"Length\":1},\"TransformationProperty\":null,\"PositionAndScaleProperty\":null,\"PositionProperty\":null},\"Children\":[]},{\"Oid\":21,\"Name\":\"Door_FL\",\"TypeClass\":{\"Name\":\"Signal\",\"Class\":3,\"SignalProperty\":{\"ObjectsCount\":1,\"InstrumentInput\":\"Input port\",\"Description\":null,\"Unit\":null,\"Type\":0,\"Length\":1},\"TransformationProperty\":null,\"PositionAndScaleProperty\":null,\"PositionProperty\":null},\"Children\":[]},{\"Oid\":22,\"Name\":\"Door_FR\",\"TypeClass\":{\"Name\":\"Signal\",\"Class\":3,\"SignalProperty\":{\"ObjectsCount\":1,\"InstrumentInput\":\"Input port\",\"Description\":null,\"Unit\":null,\"Type\":0,\"Length\":1},\"TransformationProperty\":null,\"PositionAndScaleProperty\":null,\"PositionProperty\":null},\"Children\":[]},{\"Oid\":23,\"Name\":\"Door_RL\",\"TypeClass\":{\"Name\":\"Signal\",\"Class\":3,\"SignalProperty\":{\"ObjectsCount\":1,\"InstrumentInput\":\"Input port\",\"Description\":null,\"Unit\":null,\"Type\":0,\"Length\":1},\"TransformationProperty\":null,\"PositionAndScaleProperty\":null,\"PositionProperty\":null},\"Children\":[]},{\"Oid\":24,\"Name\":\"Door_RR\",\"TypeClass\":{\"Name\":\"Signal\",\"Class\":3,\"SignalProperty\":{\"ObjectsCount\":1,\"InstrumentInput\":\"Input port\",\"Description\":null,\"Unit\":null,\"Type\":0,\"Length\":1},\"TransformationProperty\":null,\"PositionAndScaleProperty\":null,\"PositionProperty\":null},\"Children\":[]},{\"Oid\":25,\"Name\":\"Hood\",\"TypeClass\":{\"Name\":\"Signal\",\"Class\":3,\"SignalProperty\":{\"ObjectsCount\":1,\"InstrumentInput\":\"Input port\",\"Description\":null,\"Unit\":null,\"Type\":0,\"Length\":1},\"TransformationProperty\":null,\"PositionAndScaleProperty\":null,\"PositionProperty\":null},\"Children\":[]},{\"Oid\":26,\"Name\":\"Trunk\",\"TypeClass\":{\"Name\":\"Signal\",\"Class\":3,\"SignalProperty\":{\"ObjectsCount\":1,\"InstrumentInput\":\"Input port\",\"Description\":null,\"Unit\":null,\"Type\":0,\"Length\":1},\"TransformationProperty\":null,\"PositionAndScaleProperty\":null,\"PositionProperty\":null},\"Children\":[]}]}]}"  evalStr=dsmsi(gcb, 'EvalJson')  sampleTime=-1  globalBlockId=0  objectsBlockId=dsmsi(gcb, 'GetObjectBlockId')  objectsBlockGuiOpen=dsmsi(gcb, 'GetSdoGuiStatus')  dialogIsOpen=0  blockVersion=60  highPrecision=0  validNameBckp=Vehicle
      settings: SourceProductName=dSPACE MSI Blockset
  Visibility : GotoTagVisibility  GotoTag=TireRadius
  Visibility1 : GotoTagVisibility  GotoTag=Pos_z_Offset_Arrow
  Visibility2 : GotoTagVisibility  GotoTag=Scaling_F_Tire
  Visibility3 : GotoTagVisibility  GotoTag=Scaling_Fxy_Arrow
  Visibility4 : GotoTagVisibility  GotoTag=Pos_y_Offset_Arrow
  Visibility5 : GotoTagVisibility  GotoTag=Sw_TireRadius
  Wheel_FL : Subsystem
  Wheel_FR : Subsystem
  Wheel_RL : Subsystem
  Wheel_RR : Subsystem
  Chassis_Transformation_Matrix : Outport
  tag scope: Pos_y_Offset_Arrow=scoped, Pos_z_Offset_Arrow=scoped, Scaling_F_Tire=scoped, Scaling_Fxy_Arrow=scoped, Sw_TireRadius=scoped, TireRadius=scoped
  wires:
  Demux/6 -> Vehicle/48
  Demux/5 -> Vehicle/47
  Demux/4 -> Vehicle/46
  Demux/3 -> Vehicle/45
  Demux/2 -> Vehicle/44
  Demux/1 -> Vehicle/43
  TireForceRightFront/4(Scaling_R_z) -> Vehicle/29
  TireForceRightFront/3(Scaling_R_y) -> Vehicle/27
  TireForceRightFront/2(Scaling_R_x) -> Vehicle/25
  TireForceRightFront/1(Translation_R) -> Vehicle/24, Vehicle/26, Vehicle/28
  TireForceLeftFront/4(Scaling_L_z) -> Vehicle/23
  TireForceLeftFront/3(Scaling_L_y) -> Vehicle/21
  TireForceLeftFront/2(Scaling_L_x) -> Vehicle/19
  TireForceLeftFront/1(Translation_L) -> Vehicle/18, Vehicle/20, Vehicle/22
  Enable_Data_Transfer/1 -> Vehicle/1
  Wheel_RR/3(Scaling) -> Vehicle/17
  Wheel_RR/2(Rotation) -> Vehicle/16
  Wheel_RR/1(Translation) -> Vehicle/15
  Wheel_RL/3(Scaling) -> Vehicle/14
  Wheel_RL/2(Rotation) -> Vehicle/13
  Wheel_RL/1(Translation) -> Vehicle/12
  Wheel_FR/3(Scaling) -> Vehicle/11
  Wheel_FR/2(Rotation) -> Vehicle/10
  Wheel_FR/1(Translation) -> Vehicle/9
  Wheel_FL/1(Translation) -> Vehicle/6
  Wheel_FL/3(Scaling) -> Vehicle/8
  Wheel_FL/2(Rotation) -> Vehicle/7
  Steering_Wheel/2(Rotation) -> Vehicle/5
  Steering_Wheel/1(Translation) -> Vehicle/4
  Chassis/2(Rotation) -> Vehicle/3
  Chassis/1(Translation) -> Vehicle/2
  ASM_Vehicle_Lights/1 -> Vehicle/42
  TireForceLeftRear/1(Translation_L) -> Vehicle/30, Vehicle/32, Vehicle/34
  TireForceLeftRear/2(Scaling_L_x) -> Vehicle/31
  TireForceLeftRear/3(Scaling_L_y) -> Vehicle/33
  TireForceLeftRear/4(Scaling_L_z) -> Vehicle/35
  TireForceRightRear/1(Translation_R) -> Vehicle/36, Vehicle/40, Vehicle/38
  TireForceRightRear/2(Scaling_R_x) -> Vehicle/37
  TireForceRightRear/3(Scaling_R_y) -> Vehicle/39
  TireForceRightRear/4(Scaling_R_z) -> Vehicle/41
  TireRadius[m]/1 -> [TireRadius]
  Pos_y_Offset_Arrow[m]/1 -> [Pos_y_Offset_Arrow]
  Scaling_Fxy_Arrow[]/1 -> [Scaling_Fxy_Arrow]
  Pos_z_Offset_Arrow[m]/1 -> [Pos_z_Offset_Arrow]
  Sw_TireRadius[0|1]/1 -> [Sw_TireRadius]
  Scaling_F_Tire[]/1 -> [Scaling_F_Tire]
  ASM_Vehicle_Doors/1 -> Demux/1
  VehicleDynamics_Animation/1 -> Chassis/1(VehicleDynamics_Animation), Steering_Wheel/1(VehicleDynamics_Animation), Wheel_RL/1(VehicleDynamics_Animation), TireForceLeftFront/1(VehicleDynamics_Animation), TireForceRightFront/1(VehicleDynamics_Animation), TireForceLeftRear/1(VehicleDynamics_Animation), TireForceRightRear/1(VehicleDynamics_Animation), Wheel_RR/1(VehicleDynamics_Animation), Wheel_FR/1(VehicleDynamics_Animation), Wheel_FL/1(VehicleDynamics_Animation)
  Vehicle/1 -> Chassis_Transformation_Matrix/1

== system ASM_Traffic_new/AnimationInterface/ANIMATION_INTERFACE/ASM_Vehicle_Instruments ==
  VehicleDynamics_Animation : Inport
  Environment_Animation : Inport  Port=2
  Drivetrain_Animation : Inport  Port=3
  Bus Selector1 : BusSelector  OutputSignals=v_x_Vehicle_CoG[km|h],a_y_Vehicle_CoG[m|s2],YawRate_Vehicle_CoG[deg|s]
  Bus Selector15 : BusSelector  OutputSignals=n_Engine[rpm],Gear[]
  Bus Selector2 : BusSelector  OutputSignals=s_Vehicle[m],Angle_Yaw_Vehicle_CoorSys_E[deg]
  Bus Selector4 : BusSelector  OutputSignals=s_Veh_Road[m],ManeuverTime[s],ManeuverState[]
  Enable_Data_Transfer : Constant
  Vehicle_Instruments : dsmsilib/dsmsi_simulation_data_objects_BL1  Priority=10001  parameterStr="{\"Version\":1,\"TransformInput\":false,\"EnableInput\":true,\"Objects\":[{\"Oid\":1,\"Name\":\"Speed\",\"TypeClass\":{\"Name\":\"Signal\",\"Class\":3,\"SignalProperty\":{\"InstrumentInput\":\"Input port\",\"Description\":null,\"Unit\":\"km/h\",\"Type\":0,\"Length\":1,\"ObjectsCount\":1},\"TransformationProperty\":null,\"PositionAndScaleProperty\":null,\"PositionProperty\":null},\"Children\":[]},{\"Oid\":2,\"Name\":\"LatAcc\",\"TypeClass\":{\"Name\":\"Signal\",\"Class\":3,\"SignalProperty\":{\"InstrumentInput\":\"Input port\",\"Description\":null,\"Unit\":\"m/s2\",\"Type\":0,\"Length\":1,\"ObjectsCount\":1},\"TransformationProperty\":null,\"PositionAndScaleProperty\":null,\"PositionProperty\":null},\"Children\":[]},{\"Oid\":3,\"Name\":\"YawRate\",\"TypeClass\":{\"Name\":\"Signal\",\"Class\":3,\"SignalProperty\":{\"InstrumentInput\":\"Input port\",\"Description\":null,\"Unit\":\"deg/s\",\"Type\":0,\"Length\":1,\"ObjectsCount\":1},\"TransformationProperty\":null,\"PositionAndScaleProperty\":null,\"PositionProperty\":null},\"Children\":[]},{\"Oid\":4,\"Name\":\"Engine\",\"TypeClass\":{\"Name\":\"Signal\",\"Class\":3,\"SignalProperty\":{\"InstrumentInput\":\"Input port\",\"Description\":null,\"Unit\":\"rpm\",\"Type\":0,\"Length\":1,\"ObjectsCount\":1},\"TransformationProperty\":null,\"PositionAndScaleProperty\":null,\"PositionProperty\":null},\"Children\":[]},{\"Oid\":5,\"Name\":\"Gear\",\"TypeClass\":{\"Name\":\"Signal\",\"Class\":3,\"SignalProperty\":{\"InstrumentInput\":\"Input port\",\"Description\":null,\"Unit\":null,\"Type\":0,\"Length\":1,\"ObjectsCount\":1},\"TransformationProperty\":null,\"PositionAndScaleProperty\":null,\"PositionProperty\":null},\"Children\":[]},{\"Oid\":6,\"Name\":\"s_Road\",\"TypeClass\":{\"Name\":\"Signal\",\"Class\":3,\"SignalProperty\":{\"InstrumentInput\":\"Input port\",\"Description\":null,\"Unit\":\"m\",\"Type\":0,\"Length\":1,\"ObjectsCount\":1},\"TransformationProperty\":null,\"PositionAndScaleProperty\":null,\"PositionProperty\":null},\"Children\":[]},{\"Oid\":7,\"Name\":\"ManeuverTime\",\"TypeClass\":{\"Name\":\"Signal\",\"Class\":3,\"SignalProperty\":{\"InstrumentInput\":\"Input port\",\"Description\":null,\"Unit\":\"s\",\"Type\":0,\"Length\":1,\"ObjectsCount\":1},\"TransformationProperty\":null,\"PositionAndScaleProperty\":null,\"PositionProperty\":null},\"Children\":[]},{\"Oid\":8,\"Name\":\"ManeuverState\",\"TypeClass\":{\"Name\":\"Signal\",\"Class\":3,\"SignalProperty\":{\"InstrumentInput\":\"Input port\",\"Description\":null,\"Unit\":null,\"Type\":0,\"Length\":1,\"ObjectsCount\":1},\"TransformationProperty\":null,\"PositionAndScaleProperty\":null,\"PositionProperty\":null},\"Children\":[]},{\"Oid\":9,\"Name\":\"DrivenDistance\",\"TypeClass\":{\"Name\":\"Signal\",\"Class\":3,\"SignalProperty\":{\"InstrumentInput\":\"Input port\",\"Description\":null,\"Unit\":\"m\",\"Type\":0,\"Length\":1,\"ObjectsCount\":1},\"TransformationProperty\":null,\"PositionAndScaleProperty\":null,\"PositionProperty\":null},\"Children\":[]},{\"Oid\":10,\"Name\":\"YawAngle\",\"TypeClass\":{\"Name\":\"Signal\",\"Class\":3,\"SignalProperty\":{\"InstrumentInput\":\"Input port\",\"Description\":null,\"Unit\":\"deg\",\"Type\":0,\"Length\":1,\"ObjectsCount\":1},\"TransformationProperty\":null,\"PositionAndScaleProperty\":null,\"PositionProperty\":null},\"Children\":[]}]}"  evalStr=dsmsi(gcb, 'EvalJson')  sampleTime=-1  globalBlockId=0  objectsBlockId=dsmsi(gcb, 'GetObjectBlockId')  objectsBlockGuiOpen=dsmsi(gcb, 'GetSdoGuiStatus')  dialogIsOpen=0  blockVersion=60  highPrecision=0  validNameBckp=Vehicle_Instruments
      settings: SourceProductName=dSPACE MSI Blockset
  wires:
  Enable_Data_Transfer/1 -> Vehicle_Instruments/1
  Environment_Animation/1 -> Bus Selector4/1
  Bus Selector2/2 -> Vehicle_Instruments/11  "<Angle_Yaw_Vehicle_CoorSys_E[deg]>"
  Bus Selector2/1 -> Vehicle_Instruments/10  "<s_Vehicle[m]>"
  Bus Selector4/1 -> Vehicle_Instruments/7  "<s_Veh_Road[m]>"
  Bus Selector4/2 -> Vehicle_Instruments/8  "<ManeuverTime[s]>"
  Bus Selector1/2 -> Vehicle_Instruments/3  "<a_y_Vehicle_CoG[m|s2]>"
  Bus Selector1/1 -> Vehicle_Instruments/2  "<v_x_Vehicle_CoG[km|h]>"
  Bus Selector1/3 -> Vehicle_Instruments/4  "<YawRate_Vehicle_CoG[deg|s]>"
  Bus Selector4/3 -> Vehicle_Instruments/9  "<ManeuverState[]>"
  VehicleDynamics_Animation/1 -> Bus Selector1/1, Bus Selector2/1
  Drivetrain_Animation/1 -> Bus Selector15/1
  Bus Selector15/1 -> Vehicle_Instruments/5  "<n_Engine[rpm]>"
  Bus Selector15/2 -> Vehicle_Instruments/6  "<Gear[]>"
